simulink model "lab_2"  (R2025b)
settings: Solver=VariableStepAuto  StartTime=0.0  StopTime=4  RelTol=1e-3
values from neighbouring files (symbols this model uses):
  a0 = d2 - (1/tau)    [controller.m]    (also in controllerGUI.m; simulink_constants.m = 44.752429)
  a0_d = -0.914329121458805    (= -0.914329121459)    [simulink_constants.m]
  a1 = 1    [controller.m]    (also in controllerGUI.m; simulink_constants.m)
  a1_d = 1.000000    (= 1)    [simulink_constants.m]
  b0 = (tau*d0) / K1    [controller.m]    (also in controllerGUI.m; simulink_constants.m = -225.747004)
  b0_d = 2.270448497190859    (= 2.27044849719)    [simulink_constants.m]
  b1 = (tau*d1 - a0) / K1    [controller.m]    (also in controllerGUI.m; simulink_constants.m = -2.597804)
  b1_d = -2.702602561764911    (= -2.70260256176)    [simulink_constants.m]
  k1 = -(tau * (omega^2))/kp    [simulink_constants.m]
  tau = 0.02367    [controller.m]    (also in controllerCLI.m; controllerGUI.m = handles.plant.tau; simulink_constants.m = 1/(2 * zeta * omega))
settings Model: Creator=ishraqanwar  LastModifiedBy=sengu

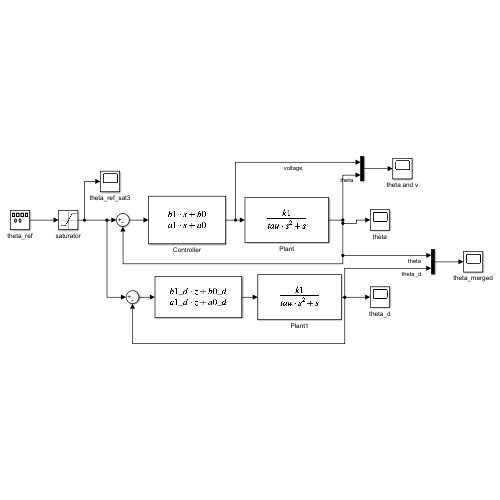
[thumbnail: Simulink's stored preview of the top-level diagram]
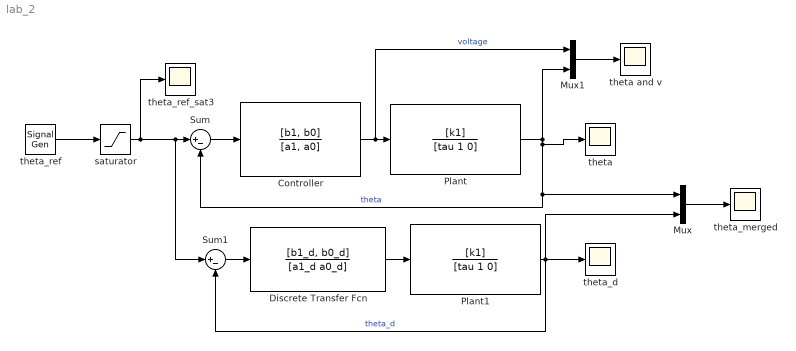
== system lab_2 ==
  Controller : TransferFcn  Numerator=[b1, b0]  Denominator=[a1, a0]
  Discrete Transfer Fcn : DiscreteTransferFcn  Numerator=[b1_d, b0_d]  Denominator=[a1_d a0_d]  SampleTime=0.002
  Mux : Mux  Inputs=2
  Mux1 : Mux  Inputs=2
  Plant : TransferFcn  Numerator=[k1]  Denominator=[tau 1 0]
  Plant1 : TransferFcn  Numerator=[k1]  Denominator=[tau 1 0]
  Sum : Sum  Inputs=|+-
  Sum1 : Sum  Inputs=|+-
  saturator : Saturate  UpperLimit=0.7  LowerLimit=-0.7
  theta : Scope
      settings: ActiveDisplayYMinimum=-1  ActiveDisplayYMaximum=1
  theta and v : Scope
      settings: MaximizeAxes=On  ActiveDisplayYMinimum=-7.5022222853958631  ActiveDisplayYMaximum=7.5022108694785  DataLoggingVariableName=ScopeData3
  theta_d : Scope
      settings: ActiveDisplayYMinimum=-0.8924001809738773  ActiveDisplayYMaximum=0.89240020720480473
  theta_merged : Scope
      settings: ActiveDisplayYMinimum=-0.96293985822614647  ActiveDisplayYMaximum=1.0195310379588949  DataLoggingVariableName=ScopeData2
  theta_ref : SignalGenerator  WaveForm=square  Amplitude=1.0  Frequency=0.5
  theta_ref_sat3 : Scope
      settings: ActiveDisplayYMinimum=-1  ActiveDisplayYMaximum=1  DataLoggingVariableName=ScopeData4
  wires:
  Plant/1 -> Mux/1, Sum/2, theta/1, Mux1/2  "theta"
  theta_ref/1 -> saturator/1
  saturator/1 -> Sum1/1, Sum/1, theta_ref_sat3/1
  Controller/1 -> Mux1/1, Plant/1  "voltage"
  Sum/1 -> Controller/1
  Plant1/1 -> Mux/2, Sum1/2, theta_d/1  "theta_d"
  Discrete Transfer Fcn/1 -> Plant1/1
  Sum1/1 -> Discrete Transfer Fcn/1
  Mux/1 -> theta_merged/1
  Mux1/1 -> theta and v/1
